simulink model "ASM_Traffic_A11"  (R2026a)
settings: Solver=ode1  StartTime=SIM.tstart.v  StopTime=SIM.tend.v  FixedStep=SIM.StepSize.v
PostLoadFcn:
  | if any(exist('dsrtsu_mdlpostloadfcn', 'file') ~= 0), dsrtsu_mdlpostloadfcn('Execute', bdroot); end
  | try, asm_mdl_postloadfcn(bdroot, 'UpdateModel', 3600); catch, disp(lasterr); end,
InitFcn:
  | , if any(exist('rtifpga_mdlclblib', 'file') ~= 0), rtifpga_mdlclblib('Init', bdroot); end,
  | , if any(exist('dsmpb_private', 'file') ~= 0), dsmpb_private('dsmpb_mdlclblib', 'Init', bdroot); end,
undefined symbols (not defined in the file): _to_, a0b2, ASM_BrakeHydraulics_DemoSystems, ASM_VehicleDynamics_DemoSystems, b98103fe8ad365046cd0, BrakeCircuit, controllerConfig, CPT, Crankshaft, DiscIntNeverNeededParam, dsmsi, FinalDriveAssembly, instance, MDL, ModeSignals, mu, Pos_BrakePedal_Maneuver, rad, RefSignals, s_to_rpm, SIM, SoftECU, Suspension, Tire, Transmission
libraries: ASM_Traffic_lib x135, simulink x98, ASM_Utils_lib x77, ASM_VehicleDynamics_lib x70, ASM_Environment_lib x22, dsmpblib x20, dsmsilib x15, MDLD_Utils_lib x10, ASM_BrakeHydraulics_lib x3, sl_discontinuities x2
(part 13 of 63)

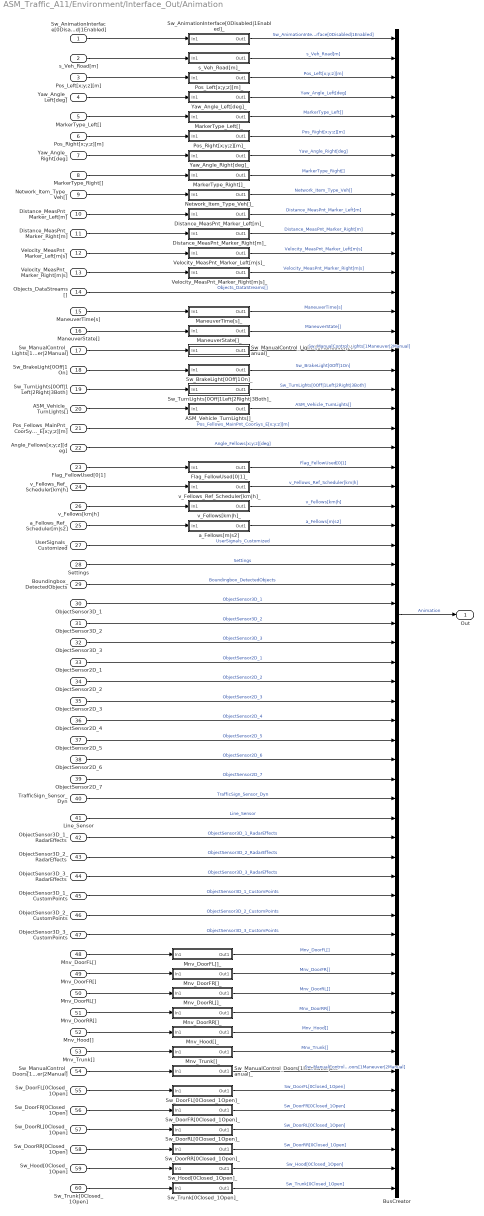
== system ASM_Traffic_A11/Environment/Interface_Out/Animation ==
  Sw_AnimationInterface[0Disabled|1Enabled] : Inport
  s_Veh_Road[m] : Inport  Port=2
  Pos_Left[x;y;z][m] : Inport  Port=3
  Yaw_Angle_Left[deg] : Inport  Port=4
  MarkerType_Left[] : Inport  Port=5
  Pos_Right[x;y;z][m] : Inport  Port=6
  Yaw_Angle_Right[deg] : Inport  Port=7
  MarkerType_Right[] : Inport  Port=8
  Network_Item_Type_Veh[] : Inport  Port=9
  Distance_MeasPnt_Marker_Left[m] : Inport  Port=10
  Distance_MeasPnt_Marker_Right[m] : Inport  Port=11
  Velocity_MeasPnt_Marker_Left[m|s] : Inport  Port=12
  Velocity_MeasPnt_Marker_Right[m|s] : Inport  Port=13
  Objects_DataStreams[] : Inport  Port=14
  ManeuverTime[s] : Inport  Port=15
  ManeuverState[] : Inport  Port=16
  Sw_ManualControl_Lights[1Maneuver|2Manual] : Inport  Port=17
  Sw_BrakeLight[0Off|1On] : Inport  Port=18
  Sw_TurnLights[0Off|1Left|2Right|3Both] : Inport  Port=19
  ASM_Vehicle_TurnLights[] : Inport  Port=20
  Pos_Fellows_MainPnt_CoorSys_E[x;y;z][m] : Inport  Port=21
  Angle_Fellows[x;y;z][deg] : Inport  Port=22
  Flag_FellowUsed[0|1] : Inport  Port=23
  v_Fellows_Ref_Scheduler[km|h] : Inport  Port=24
  a_Fellows_Ref_Scheduler[m|s2] : Inport  Port=25
  v_Fellows[km|h] : Inport  Port=26
  UserSignals_Customized : Inport  Port=27
  Settings : Inport  Port=28
  Boundingbox_DetectedObjects : Inport  Port=29
  ObjectSensor3D_1 : Inport  Port=30
  ObjectSensor3D_2 : Inport  Port=31
  ObjectSensor3D_3 : Inport  Port=32
  ObjectSensor2D_1 : Inport  Port=33
  ObjectSensor2D_2 : Inport  Port=34
  ObjectSensor2D_3 : Inport  Port=35
  ObjectSensor2D_4 : Inport  Port=36
  ObjectSensor2D_5 : Inport  Port=37
  ObjectSensor2D_6 : Inport  Port=38
  ObjectSensor2D_7 : Inport  Port=39
  TrafficSign_Sensor_Dyn : Inport  Port=40
  Line_Sensor : Inport  Port=41
  ObjectSensor3D_1_RadarEffects : Inport  Port=42
  ObjectSensor3D_2_RadarEffects : Inport  Port=43
  ObjectSensor3D_3_RadarEffects : Inport  Port=44
  ObjectSensor3D_1_CustomPoints : Inport  Port=45
  ObjectSensor3D_2_CustomPoints : Inport  Port=46
  ObjectSensor3D_3_CustomPoints : Inport  Port=47
  Mnv_DoorFL[] : Inport  Port=48
  Mnv_DoorFR[] : Inport  Port=49
  Mnv_DoorRL[] : Inport  Port=50
  Mnv_DoorRR[] : Inport  Port=51
  Mnv_Hood[] : Inport  Port=52
  Mnv_Trunk[] : Inport  Port=53
  Sw_ManualControl_Doors[1Maneuver|2Manual] : Inport  Port=54
  Sw_DoorFL[0Closed_1Open] : Inport  Port=55
  Sw_DoorFR[0Closed_1Open] : Inport  Port=56
  Sw_DoorRL[0Closed_1Open] : Inport  Port=57
  Sw_DoorRR[0Closed_1Open] : Inport  Port=58
  Sw_Hood[0Closed_1Open] : Inport  Port=59
  Sw_Trunk[0Closed_1Open] : Inport  Port=60
  ASM_Vehicle_TurnLights[]_ : Subsystem
      mask Display: disp('')
  BusCreator : BusCreator  Inputs=60
  Distance_MeasPnt_Marker_Left[m]_ : Subsystem
      mask Display: disp('')
  Distance_MeasPnt_Marker_Right[m]_ : Subsystem
      mask Display: disp('')
  Flag_FellowUsed[0|1]_ : Subsystem
      mask Display: disp('')
  ManeuverState[]_ : Subsystem
      mask Display: disp('')
  ManeuverTime[s]_ : Subsystem
      mask Display: disp('')
  MarkerType_Left[]_ : Subsystem
      mask Display: disp('')
  MarkerType_Right[]_ : Subsystem
      mask Display: disp('')
  Mnv_DoorFL[]_ : Subsystem
      mask Display: disp('')
  Mnv_DoorFR[]_ : Subsystem
      mask Display: disp('')
  Mnv_DoorRL[]_ : Subsystem
      mask Display: disp('')
  Mnv_DoorRR[]_ : Subsystem
      mask Display: disp('')
  Mnv_Hood[]_ : Subsystem
      mask Display: disp('')
  Mnv_Trunk[]_ : Subsystem
      mask Display: disp('')
  Network_Item_Type_Veh[]_ : Subsystem
      mask Display: disp('')
  Pos_Left[x;y;z][m]_ : Subsystem
      mask Display: disp('')
  Pos_Right[x;y;z][m]_ : Subsystem
      mask Display: disp('')
  Sw_AnimationInterface[0Disabled|1Enabled]_ : Subsystem
      mask Display: disp('')
  Sw_BrakeLight[0Off|1On]_ : Subsystem
      mask Display: disp('')
  Sw_DoorFL[0Closed_1Open]_ : Subsystem
      mask Display: disp('')
  Sw_DoorFR[0Closed_1Open]_ : Subsystem
      mask Display: disp('')
  Sw_DoorRL[0Closed_1Open]_ : Subsystem
      mask Display: disp('')
  Sw_DoorRR[0Closed_1Open]_ : Subsystem
      mask Display: disp('')
  Sw_Hood[0Closed_1Open]_ : Subsystem
      mask Display: disp('')
  Sw_ManualControl_Doors[1Maneuver|2Manual]_ : Subsystem
      mask Display: disp('')
  Sw_ManualControl_Lights[1Maneuver|2Manual]_ : Subsystem
      mask Display: disp('')
  Sw_Trunk[0Closed_1Open]_ : Subsystem
      mask Display: disp('')
  Sw_TurnLights[0Off|1Left|2Right|3Both]_ : Subsystem
      mask Display: disp('')
  Velocity_MeasPnt_Marker_Left[m|s]_ : Subsystem
      mask Display: disp('')
  Velocity_MeasPnt_Marker_Right[m|s]_ : Subsystem
      mask Display: disp('')
  Yaw_Angle_Left[deg]_ : Subsystem
      mask Display: disp('')
  Yaw_Angle_Right[deg]_ : Subsystem
      mask Display: disp('')
  a_Fellows[m|s2] : Subsystem
      mask Display: disp('')
  s_Veh_Road[m]_ : Subsystem
      mask Display: disp('')
  v_Fellows[km|h]_ : Subsystem
      mask Display: disp('')
  v_Fellows_Ref_Scheduler[km|h]_ : Subsystem
      mask Display: disp('')
  Out : Outport  VectorParamsAs1DForOutWhenUnconnected=off
  wires:
  Sw_AnimationInterface[0Disabled|1Enabled]_/1(Out1) -> BusCreator/1  "Sw_AnimationInterface[0Disabled|1Enabled]"
  Sw_AnimationInterface[0Disabled|1Enabled]/1 -> Sw_AnimationInterface[0Disabled|1Enabled]_/1(In1)
  a_Fellows[m|s2]/1(Out1) -> BusCreator/26  "a_Fellows[m|s2]"
  a_Fellows_Ref_Scheduler[m|s2]/1 -> a_Fellows[m|s2]/1(In1)
  ObjectSensor2D_1/1 -> BusCreator/33  "ObjectSensor2D_1"
  ObjectSensor2D_2/1 -> BusCreator/34  "ObjectSensor2D_2"
  ObjectSensor3D_1/1 -> BusCreator/30  "ObjectSensor3D_1"
  ObjectSensor2D_3/1 -> BusCreator/35  "ObjectSensor2D_3"
  ObjectSensor3D_2/1 -> BusCreator/31  "ObjectSensor3D_2"
  ObjectSensor2D_6/1 -> BusCreator/38  "ObjectSensor2D_6"
  ObjectSensor2D_4/1 -> BusCreator/36  "ObjectSensor2D_4"
  ObjectSensor2D_7/1 -> BusCreator/39  "ObjectSensor2D_7"
  TrafficSign_Sensor_Dyn/1 -> BusCreator/40  "TrafficSign_Sensor_Dyn"
  ObjectSensor3D_3_CustomPoints/1 -> BusCreator/47  "ObjectSensor3D_3_CustomPoints"
  ObjectSensor3D_3/1 -> BusCreator/32  "ObjectSensor3D_3"
  ObjectSensor3D_1_RadarEffects/1 -> BusCreator/42  "ObjectSensor3D_1_RadarEffects"
  ObjectSensor3D_3_RadarEffects/1 -> BusCreator/44  "ObjectSensor3D_3_RadarEffects"
  ObjectSensor3D_2_CustomPoints/1 -> BusCreator/46  "ObjectSensor3D_2_CustomPoints"
  ObjectSensor2D_5/1 -> BusCreator/37  "ObjectSensor2D_5"
  Line_Sensor/1 -> BusCreator/41  "Line_Sensor"
  ObjectSensor3D_1_CustomPoints/1 -> BusCreator/45  "ObjectSensor3D_1_CustomPoints"
  ObjectSensor3D_2_RadarEffects/1 -> BusCreator/43  "ObjectSensor3D_2_RadarEffects"
  Boundingbox_DetectedObjects/1 -> BusCreator/29  "Boundingbox_DetectedObjects"
  v_Fellows[km|h]_/1(Out1) -> BusCreator/25  "v_Fellows[km|h]"
  v_Fellows_Ref_Scheduler[km|h]_/1(Out1) -> BusCreator/24  "v_Fellows_Ref_Scheduler[km|h]"
  Flag_FellowUsed[0|1]_/1(Out1) -> BusCreator/23  "Flag_FellowUsed[0|1]"
  Pos_Fellows_MainPnt_CoorSys_E[x;y;z][m]/1 -> BusCreator/21  "Pos_Fellows_MainPnt_CoorSys_E[x;y;z][m]"
  Settings/1 -> BusCreator/28  "Settings"
  v_Fellows_Ref_Scheduler[km|h]/1 -> v_Fellows_Ref_Scheduler[km|h]_/1(In1)
  UserSignals_Customized/1 -> BusCreator/27  "UserSignals_Customized"
  Angle_Fellows[x;y;z][deg]/1 -> BusCreator/22  "Angle_Fellows[x;y;z][deg]"
  v_Fellows[km|h]/1 -> v_Fellows[km|h]_/1(In1)
  Flag_FellowUsed[0|1]/1 -> Flag_FellowUsed[0|1]_/1(In1)
  ASM_Vehicle_TurnLights[]_/1(Out1) -> BusCreator/20  "ASM_Vehicle_TurnLights[]"
  Sw_TurnLights[0Off|1Left|2Right|3Both]_/1(Out1) -> BusCreator/19  "Sw_TurnLights[0Off|1Left|2Right|3Both]"
  Sw_BrakeLight[0Off|1On]_/1(Out1) -> BusCreator/18  "Sw_BrakeLight[0Off|1On]"
  Sw_ManualControl_Lights[1Maneuver|2Manual]_/1(Out1) -> BusCreator/17  "Sw_ManualControl_Lights[1Maneuver|2Manual]"
  ManeuverState[]_/1(Out1) -> BusCreator/16  "ManeuverState[]"
  ManeuverTime[s]_/1(Out1) -> BusCreator/15  "ManeuverTime[s]"
  ManeuverState[]/1 -> ManeuverState[]_/1(In1)
  Sw_BrakeLight[0Off|1On]/1 -> Sw_BrakeLight[0Off|1On]_/1(In1)
  ManeuverTime[s]/1 -> ManeuverTime[s]_/1(In1)
  Sw_TurnLights[0Off|1Left|2Right|3Both]/1 -> Sw_TurnLights[0Off|1Left|2Right|3Both]_/1(In1)
  Sw_ManualControl_Lights[1Maneuver|2Manual]/1 -> Sw_ManualControl_Lights[1Maneuver|2Manual]_/1(In1)
  ASM_Vehicle_TurnLights[]/1 -> ASM_Vehicle_TurnLights[]_/1(In1)
  Objects_DataStreams[]/1 -> BusCreator/14  "Objects_DataStreams[]"
  Velocity_MeasPnt_Marker_Right[m|s]_/1(Out1) -> BusCreator/13  "Velocity_MeasPnt_Marker_Right[m|s]"
  Velocity_MeasPnt_Marker_Left[m|s]_/1(Out1) -> BusCreator/12  "Velocity_MeasPnt_Marker_Left[m|s]"
  Distance_MeasPnt_Marker_Right[m]_/1(Out1) -> BusCreator/11  "Distance_MeasPnt_Marker_Right[m]"
  Distance_MeasPnt_Marker_Left[m]_/1(Out1) -> BusCreator/10  "Distance_MeasPnt_Marker_Left[m]"
  Network_Item_Type_Veh[]_/1(Out1) -> BusCreator/9  "Network_Item_Type_Veh[]"
  MarkerType_Right[]_/1(Out1) -> BusCreator/8  "MarkerType_Right[]"
  Yaw_Angle_Right[deg]_/1(Out1) -> BusCreator/7  "Yaw_Angle_Right[deg]"
  Pos_Right[x;y;z][m]_/1(Out1) -> BusCreator/6  "Pos_Right[x;y;z][m]"
  MarkerType_Left[]_/1(Out1) -> BusCreator/5  "MarkerType_Left[]"
  Yaw_Angle_Left[deg]_/1(Out1) -> BusCreator/4  "Yaw_Angle_Left[deg]"
  Pos_Left[x;y;z][m]_/1(Out1) -> BusCreator/3  "Pos_Left[x;y;z][m]"
  s_Veh_Road[m]_/1(Out1) -> BusCreator/2  "s_Veh_Road[m]"
  s_Veh_Road[m]/1 -> s_Veh_Road[m]_/1(In1)
  Pos_Left[x;y;z][m]/1 -> Pos_Left[x;y;z][m]_/1(In1)
  Pos_Right[x;y;z][m]/1 -> Pos_Right[x;y;z][m]_/1(In1)
  Yaw_Angle_Left[deg]/1 -> Yaw_Angle_Left[deg]_/1(In1)
  Distance_MeasPnt_Marker_Right[m]/1 -> Distance_MeasPnt_Marker_Right[m]_/1(In1)
  MarkerType_Left[]/1 -> MarkerType_Left[]_/1(In1)
  MarkerType_Right[]/1 -> MarkerType_Right[]_/1(In1)
  Yaw_Angle_Right[deg]/1 -> Yaw_Angle_Right[deg]_/1(In1)
  Velocity_MeasPnt_Marker_Right[m|s]/1 -> Velocity_MeasPnt_Marker_Right[m|s]_/1(In1)
  Network_Item_Type_Veh[]/1 -> Network_Item_Type_Veh[]_/1(In1)
  Velocity_MeasPnt_Marker_Left[m|s]/1 -> Velocity_MeasPnt_Marker_Left[m|s]_/1(In1)
  Distance_MeasPnt_Marker_Left[m]/1 -> Distance_MeasPnt_Marker_Left[m]_/1(In1)
  BusCreator/1 -> Out/1  "Animation"
  Mnv_Trunk[]/1 -> Mnv_Trunk[]_/1(In1)
  Mnv_DoorFR[]/1 -> Mnv_DoorFR[]_/1(In1)
  Mnv_Hood[]/1 -> Mnv_Hood[]_/1(In1)
  Mnv_DoorRL[]/1 -> Mnv_DoorRL[]_/1(In1)
  Mnv_DoorRR[]/1 -> Mnv_DoorRR[]_/1(In1)
  Mnv_DoorFL[]_/1(Out1) -> BusCreator/48  "Mnv_DoorFL[]"
  Mnv_DoorFL[]/1 -> Mnv_DoorFL[]_/1(In1)
  Mnv_DoorFR[]_/1(Out1) -> BusCreator/49  "Mnv_DoorFR[]"
  Mnv_DoorRL[]_/1(Out1) -> BusCreator/50  "Mnv_DoorRL[]"
  Mnv_DoorRR[]_/1(Out1) -> BusCreator/51  "Mnv_DoorRR[]"
  Mnv_Hood[]_/1(Out1) -> BusCreator/52  "Mnv_Hood[]"
  Mnv_Trunk[]_/1(Out1) -> BusCreator/53  "Mnv_Trunk[]"
  Sw_DoorFL[0Closed_1Open]_/1(Out1) -> BusCreator/55  "Sw_DoorFL[0Closed_1Open]"
  Sw_DoorFR[0Closed_1Open]_/1(Out1) -> BusCreator/56  "Sw_DoorFR[0Closed_1Open]"
  Sw_ManualControl_Doors[1Maneuver|2Manual]_/1(Out1) -> BusCreator/54  "Sw_ManualControl_Doors[1Maneuver|2Manual]"
  Sw_Hood[0Closed_1Open]_/1(Out1) -> BusCreator/59  "Sw_Hood[0Closed_1Open]"
  Sw_DoorRR[0Closed_1Open]_/1(Out1) -> BusCreator/58  "Sw_DoorRR[0Closed_1Open]"
  Sw_DoorRL[0Closed_1Open]_/1(Out1) -> BusCreator/57  "Sw_DoorRL[0Closed_1Open]"
  Sw_Trunk[0Closed_1Open]_/1(Out1) -> BusCreator/60  "Sw_Trunk[0Closed_1Open]"
  Sw_ManualControl_Doors[1Maneuver|2Manual]/1 -> Sw_ManualControl_Doors[1Maneuver|2Manual]_/1(In1)
  Sw_DoorFL[0Closed_1Open]/1 -> Sw_DoorFL[0Closed_1Open]_/1(In1)
  Sw_DoorFR[0Closed_1Open]/1 -> Sw_DoorFR[0Closed_1Open]_/1(In1)
  Sw_DoorRL[0Closed_1Open]/1 -> Sw_DoorRL[0Closed_1Open]_/1(In1)
  Sw_DoorRR[0Closed_1Open]/1 -> Sw_DoorRR[0Closed_1Open]_/1(In1)
  Sw_Hood[0Closed_1Open]/1 -> Sw_Hood[0Closed_1Open]_/1(In1)
  Sw_Trunk[0Closed_1Open]/1 -> Sw_Trunk[0Closed_1Open]_/1(In1)

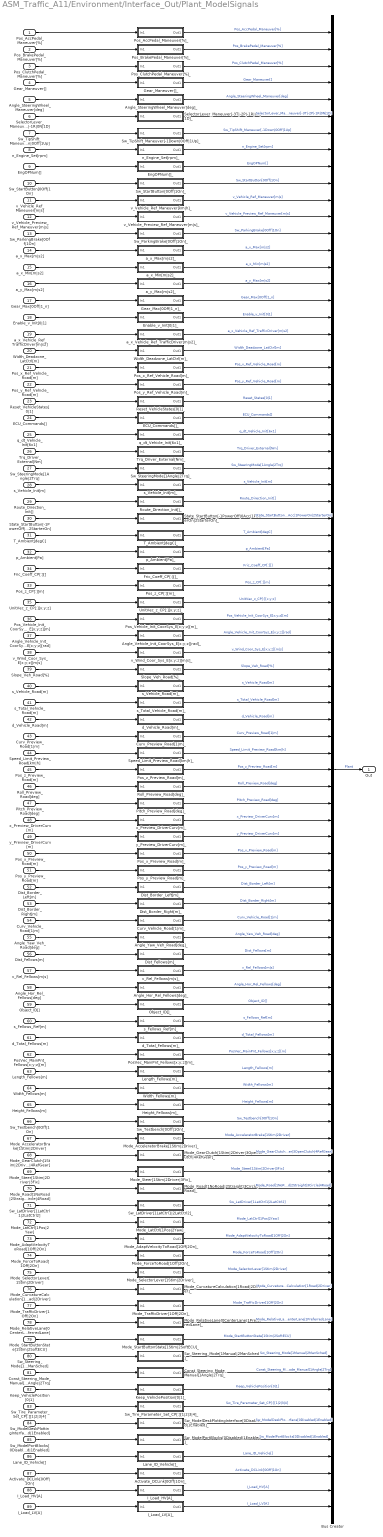
== system ASM_Traffic_A11/Environment/Interface_Out/Plant_ModelSignals ==
  Pos_AccPedal_Maneuver[%] : Inport
  Pos_BrakePedal_Maneuver[%] : Inport  Port=2
  Pos_ClutchPedal_Maneuver[%] : Inport  Port=3
  Gear_Maneuver[] : Inport  Port=4
  Angle_SteeringWheel_Maneuver[deg] : Inport  Port=5
  SelectorLever_Maneuver[-3T|-2P|-1R|0N|1D] : Inport  Port=6
  Sw_TipShift_Maneuver[-1Down|0Off|1Up] : Inport  Port=7
  n_Engine_Set[rpm] : Inport  Port=8
  EngOPNum[] : Inport  Port=9
  Sw_StartButton[0Off|1On] : Inport  Port=10
  v_Vehicle_Ref_Maneuver[m|s] : Inport  Port=11
  v_Vehicle_Preview_Ref_Maneuver[m|s] : Inport  Port=12
  Sw_ParkingBrake[0Off|1On] : Inport  Port=13
  a_x_Max[m|s2] : Inport  Port=14
  a_x_Min[m|s2] : Inport  Port=15
  a_y_Max[m|s2] : Inport  Port=16
  Gear_Max[0Off|1_n] : Inport  Port=17
  Enable_v_Init[0|1] : Inport  Port=18
  a_x_Vehicle_Ref_TrafficDriver[m|s2] : Inport  Port=19
  Width_Deadzone_LatCtrl[m] : Inport  Port=20
  Pos_x_Ref_Vehicle_Road[m] : Inport  Port=21
  Pos_y_Ref_Vehicle_Road[m] : Inport  Port=22
  Reset_VehicleStates[0|1] : Inport  Port=23
  ECU_Commands[] : Inport  Port=24
  q_dt_Vehicle_Init[6x1] : Inport  Port=25
  Trq_Driver_External[Nm] : Inport  Port=26
  Sw_SteeringMode[1Angle|2Trq] : Inport  Port=27
  s_Vehicle_Init[m] : Inport  Port=28
  Route_Direction_Init[] : Inport  Port=29
  State_StartButton[-1PowerOff|0Acc|1PowerOn|2StarterOn] : Inport  Port=30
  T_Ambient[degC] : Inport  Port=31
  p_Ambient[Pa] : Inport  Port=32
  Pos_z_CP[:][m] : Inport  Port=33
  Fric_Coeff_CP[:][] : Inport  Port=34
  UnitVec_z_CP[:][x;y;z] : Inport  Port=35
  Pos_Vehicle_Init_CoorSys_E[x;y;z][m] : Inport  Port=36
  Angle_Vehicle_Init_CoorSys_E[x;y;z][rad] : Inport  Port=37
  v_Wind_Coor_Sys_E[x;y;z][m|s] : Inport  Port=38
  Slope_Veh_Road[%] : Inport  Port=39
  s_Vehicle_Road[m] : Inport  Port=40
  s_Total_Vehicle_Road[m] : Inport  Port=41
  d_Vehicle_Road[m] : Inport  Port=42
  Curv_Preview_Road[1|m] : Inport  Port=43
  Speed_Limit_Preview_Road[km|h] : Inport  Port=44
  Pos_z_Preview_Road[m] : Inport  Port=45
  Roll_Preview_Road[deg] : Inport  Port=46
  Pitch_Preview_Road[deg] : Inport  Port=47
  x_Preview_DriverCurv[m] : Inport  Port=48
  y_Preview_DriverCurv[m] : Inport  Port=49
  Pos_x_Preview_Road[m] : Inport  Port=50
  Pos_y_Preview_Road[m] : Inport  Port=51
  Dist_Border_Left[m] : Inport  Port=52
  Dist_Border_Right[m] : Inport  Port=53
  Curv_Vehicle_Road[1|m] : Inport  Port=54
  Angle_Yaw_Veh_Road[deg] : Inport  Port=55
  Dist_Fellows[m] : Inport  Port=56
  v_Rel_Fellows[m|s] : Inport  Port=57
  Angle_Hor_Rel_Fellows[deg] : Inport  Port=58
  Object_ID[] : Inport  Port=59
  s_Fellows_Ref[m] : Inport  Port=60
  d_Total_Fellows[m] : Inport  Port=61
  PosVec_MainPnt_Fellows[x;y;z][m] : Inport  Port=62
  Length_Fellows[m] : Inport  Port=63
  Width_Fellows[m] : Inport  Port=64
  Height_Fellows[m] : Inport  Port=65
  Sw_Testbench[0Off|1On] : Inport  Port=66
  Mode_AcceleratorBrake[1Stim|2Driver] : Inport  Port=67
  Mode_GearClutch[1Stim|2Driver|3OpenClutch|4RefGear] : Inport  Port=68
  Mode_Steer[1Stim|2Driver|3Fix] : Inport  Port=69
  Mode_Road[1NoRoad|2Straight|3Circle|4Road] : Inport  Port=70
  Sw_LatDriver[1LatCtrl1|2LatCtrl2] : Inport  Port=71
  Mode_LatCtrl[1Pos|2Yaw] : Inport  Port=72
  Mode_AdaptVelocityToRoad[1Off|2On] : Inport  Port=73
  Mode_ForceToRoad[1Off|2On] : Inport  Port=74
  Mode_SelectorLever[1Stim|2Driver] : Inport  Port=75
  Mode_CurvatureCalculation[1Road|2Driver] : Inport  Port=76
  Mode_TrafficDriver[1Off|2On] : Inport  Port=77
  Mode_RelativeLane[0CenterLane|1PreferredLane] : Inport  Port=78
  Mode_StartButtonState[1Stim|2SoftECU] : Inport  Port=79
  Sw_Steering_Mode[1Manual|2ManSched] : Inport  Port=80
  Const_Steering_Mode_Manual[1Angle|2Trq] : Inport  Port=81
  Keep_VehiclePosition[0|1] : Inport  Port=82
  Sw_Tire_Parameter_Set_CP[:][1|2|3|4] : Inport  Port=83
  Sw_ModelDeskPlottingInterface[0Disabled|1Enabled] : Inport  Port=84
  Sw_ModelPortBlocks[0Disabled|1Enabled] : Inport  Port=85
  Lane_ID_Vehicle[] : Inport  Port=86
  Activate_DCLink[0Off|1On] : Inport  Port=87
  I_Load_HV[A] : Inport  Port=88
  I_Load_LV[A] : Inport  Port=89
  Activate_DCLink[0Off|1On]_ : Subsystem
      mask Display: disp('')
  Angle_Hor_Rel_Fellows[deg]_ : Subsystem
      mask Display: disp('')
  Angle_SteeringWheel_Maneuver[deg]_ : Subsystem
      mask Display: disp('')
  Angle_Vehicle_Init_CoorSys_E[x;y;z][rad]_ : Subsystem
      mask Display: disp('')
  Angle_Yaw_Veh_Road[deg]_ : Subsystem
      mask Display: disp('')
  Bus Creator : BusCreator  Inputs=89
  Const_Steering_Mode_Manual[1Angle|2Trq]_ : Subsystem
      mask Display: disp('')
  Curv_Preview_Road[1|m]_ : Subsystem
      mask Display: disp('')
  Curv_Vehicle_Road[1|m]_ : Subsystem
      mask Display: disp('')
  Dist_Border_Left[m]_ : Subsystem
      mask Display: disp('')
  Dist_Border_Right[m]_ : Subsystem
      mask Display: disp('')
  Dist_Fellows[m]_ : Subsystem
      mask Display: disp('')
  ECU_Commands[]_ : Subsystem
      mask Display: disp('')
  Enable_v_Init[0|1]_ : Subsystem
      mask Display: disp('')
  EngOPNum[]_ : Subsystem
      mask Display: disp('')
  Fric_Coeff_CP[:][]_ : Subsystem
      mask Display: disp('')
  Gear_Maneuver[]_ : Subsystem
      mask Display: disp('')
  Gear_Max[0Off|1_n]_ : Subsystem
      mask Display: disp('')
  Height_Fellows[m]_ : Subsystem
      mask Display: disp('')
  I_Load_HV[A]_ : Subsystem
      mask Display: disp('')
  I_Load_LV[A]_ : Subsystem
      mask Display: disp('')
  Keep_VehiclePosition[0|1]_ : Subsystem
      mask Display: disp('')
  Lane_ID_Vehicle[]_ : Subsystem
      mask Display: disp('')
  Length_Fellows[m]_ : Subsystem
      mask Display: disp('')
  Mode_AcceleratorBrake[1Stim|2Driver]_ : Subsystem
      mask Display: disp('')
  Mode_AdaptVelocityToRoad[1Off|2On]_ : Subsystem
      mask Display: disp('')
  Mode_CurvatureCalculation[1Road|2Driver]_ : Subsystem
      mask Display: disp('')
  Mode_ForceToRoad[1Off|2On]_ : Subsystem
      mask Display: disp('')
  Mode_GearClutch[1Stim|2Driver|3OpenClutch|4RefGear]_ : Subsystem
      mask Display: disp('')
  Mode_LatCtrl[1Pos|2Yaw]_ : Subsystem
      mask Display: disp('')
  Mode_RelativeLane[0CenterLane|1PreferredLane]_ : Subsystem
      mask Display: disp('')
  Mode_Road[1NoRoad|2Straight|3Circle|4Road]_ : Subsystem
      mask Display: disp('')
  Mode_SelectorLever[1Stim|2Driver]_ : Subsystem
      mask Display: disp('')
  Mode_StartButtonState[1Stim|2SoftECU]_ : Subsystem
      mask Display: disp('')
  Mode_Steer[1Stim|2Driver|3Fix]_ : Subsystem
      mask Display: disp('')
  Mode_TrafficDriver[1Off|2On]_ : Subsystem
      mask Display: disp('')
  Object_ID[]_ : Subsystem
      mask Display: disp('')
  Pitch_Preview_Road[deg]_ : Subsystem
      mask Display: disp('')
  PosVec_MainPnt_Fellows[x;y;z][m]_ : Subsystem
      mask Display: disp('')
  Pos_AccPedal_Maneuver[%]_ : Subsystem
      mask Display: disp('')
  Pos_BrakePedal_Maneuver[%]_ : Subsystem
      mask Display: disp('')
  Pos_ClutchPedal_Maneuver[%]_ : Subsystem
      mask Display: disp('')
  Pos_Vehicle_Init_CoorSys_E[x;y;z][m]_ : Subsystem
      mask Display: disp('')
  Pos_x_Preview_Road[m]_ : Subsystem
      mask Display: disp('')
  Pos_x_Ref_Vehicle_Road[m]_ : Subsystem
      mask Display: disp('')
  Pos_y_Preview_Road[m]_ : Subsystem
      mask Display: disp('')
  Pos_y_Ref_Vehicle_Road[m]_ : Subsystem
      mask Display: disp('')
  Pos_z_CP[:][m]_ : Subsystem
      mask Display: disp('')
  Pos_z_Preview_Road[m]_ : Subsystem
      mask Display: disp('')
  Reset_VehicleStates[0|1]_ : Subsystem
      mask Display: disp('')
  Roll_Preview_Road[deg]_ : Subsystem
      mask Display: disp('')
  Route_Direction_Init[]_ : Subsystem
      mask Display: disp('')
  SelectorLever_Maneuver[-3T|-2P|-1R|0N|1D]_ : Subsystem
      mask Display: disp('')
  Slope_Veh_Road[%]_ : Subsystem
      mask Display: disp('')
  Speed_Limit_Preview_Road[km|h]_ : Subsystem
      mask Display: disp('')
  State_StartButton[-1PowerOff|0Acc|1PowerOn|2StarterOn]_ : Subsystem
      mask Display: disp('')
  Sw_LatDriver[1LatCtrl1|2LatCtrl2]_ : Subsystem
      mask Display: disp('')
  Sw_ModelDeskPlottingInterface[0Disabled|1Enabled]_ : Subsystem
      mask Display: disp('')
  Sw_ModelPortBlocks[0Disabled|1Enabled]_ : Subsystem
      mask Display: disp('')
  Sw_ParkingBrake[0Off|1On]_ : Subsystem
      mask Display: disp('')
  Sw_StartButton[0Off|1On]_ : Subsystem
      mask Display: disp('')
  Sw_SteeringMode[1Angle|2Trq]_ : Subsystem
      mask Display: disp('')
  Sw_Steering_Mode[1Manual|2ManSched]_ : Subsystem
      mask Display: disp('')
  Sw_Testbench[0Off|1On]_ : Subsystem
      mask Display: disp('')
  Sw_TipShift_Maneuver[-1Down|0Off|1Up]_ : Subsystem
      mask Display: disp('')
  Sw_Tire_Parameter_Set_CP[:][1|2|3|4]_ : Subsystem
      mask Display: disp('')
  T_Ambient[degC]_ : Subsystem
      mask Display: disp('')
  Trq_Driver_External[Nm]_ : Subsystem
      mask Display: disp('')
  UnitVec_z_CP[:][x;y;z]_ : Subsystem
      mask Display: disp('')
  Width_Deadzone_LatCtrl[m]_ : Subsystem
      mask Display: disp('')
  Width_Fellows[m]_ : Subsystem
      mask Display: disp('')
  a_x_Max[m|s2]_ : Subsystem
      mask Display: disp('')
  a_x_Min[m|s2]_ : Subsystem
      mask Display: disp('')
  a_x_Vehicle_Ref_TrafficDriver[m|s2]_ : Subsystem
      mask Display: disp('')
  a_y_Max[m|s2]_ : Subsystem
      mask Display: disp('')
  d_Total_Fellows[m]_ : Subsystem
      mask Display: disp('')
  d_Vehicle_Road[m]_ : Subsystem
      mask Display: disp('')
  n_Engine_Set[rpm]_ : Subsystem
      mask Display: disp('')
  p_Ambient[Pa]_ : Subsystem
      mask Display: disp('')
  q_dt_Vehicle_Init[6x1]_ : Subsystem
      mask Display: disp('')
  s_Fellows_Ref[m]_ : Subsystem
      mask Display: disp('')
  s_Total_Vehicle_Road[m]_ : Subsystem
      mask Display: disp('')
  s_Vehicle_Init[m]_ : Subsystem
      mask Display: disp('')
  s_Vehicle_Road[m]_ : Subsystem
      mask Display: disp('')
  v_Rel_Fellows[m|s]_ : Subsystem
      mask Display: disp('')
  v_Vehicle_Preview_Ref_Maneuver[m|s]_ : Subsystem
      mask Display: disp('')
  v_Vehicle_Ref_Maneuver[km|h]_ : Subsystem
      mask Display: disp('')
  v_Wind_Coor_Sys_E[x;y;z][m|s]_ : Subsystem
      mask Display: disp('')
  x_Preview_DriverCurv[m]_ : Subsystem
      mask Display: disp('')
  y_Preview_DriverCurv[m]_ : Subsystem
      mask Display: disp('')
  Out : Outport  VectorParamsAs1DForOutWhenUnconnected=off
  wires:
  Lane_ID_Vehicle[]_/1(Out1) -> Bus Creator/86  "Lane_ID_Vehicle[]"
  Lane_ID_Vehicle[]/1 -> Lane_ID_Vehicle[]_/1(In1)
  Sw_ModelDeskPlottingInterface[0Disabled|1Enabled]/1 -> Sw_ModelDeskPlottingInterface[0Disabled|1Enabled]_/1(In1)
  Sw_ModelDeskPlottingInterface[0Disabled|1Enabled]_/1(Out1) -> Bus Creator/84  "Sw_ModelDeskPlottingInterface[0Disabled|1Enabled]"
  Sw_ModelPortBlocks[0Disabled|1Enabled]/1 -> Sw_ModelPortBlocks[0Disabled|1Enabled]_/1(In1)
  Sw_ModelPortBlocks[0Disabled|1Enabled]_/1(Out1) -> Bus Creator/85  "Sw_ModelPortBlocks[0Disabled|1Enabled]"
  Bus Creator/1 -> Out/1  "Plant"
  Enable_v_Init[0|1]_/1(Out1) -> Bus Creator/18  "Enable_v_Init[0|1]"
  Enable_v_Init[0|1]/1 -> Enable_v_Init[0|1]_/1(In1)
  SelectorLever_Maneuver[-3T|-2P|-1R|0N|1D]/1 -> SelectorLever_Maneuver[-3T|-2P|-1R|0N|1D]_/1(In1)
  Sw_StartButton[0Off|1On]/1 -> Sw_StartButton[0Off|1On]_/1(In1)
  Gear_Max[0Off|1_n]/1 -> Gear_Max[0Off|1_n]_/1(In1)
  v_Vehicle_Preview_Ref_Maneuver[m|s]_/1(Out1) -> Bus Creator/12  "v_Vehicle_Preview_Ref_Maneuver[m|s]"
  v_Vehicle_Ref_Maneuver[km|h]_/1(Out1) -> Bus Creator/11  "v_Vehicle_Ref_Maneuver[m|s]"
  Pos_x_Ref_Vehicle_Road[m]/1 -> Pos_x_Ref_Vehicle_Road[m]_/1(In1)
  Gear_Max[0Off|1_n]_/1(Out1) -> Bus Creator/17  "Gear_Max[0Off|1_n]"
  Sw_StartButton[0Off|1On]_/1(Out1) -> Bus Creator/10  "Sw_StartButton[0Off|1On]"
  EngOPNum[]/1 -> EngOPNum[]_/1(In1)
  Sw_TipShift_Maneuver[-1Down|0Off|1Up]_/1(Out1) -> Bus Creator/7  "Sw_TipShift_Maneuver[-1Down|0Off|1Up]"
  n_Engine_Set[rpm]/1 -> n_Engine_Set[rpm]_/1(In1)
  Pos_BrakePedal_Maneuver[%]_/1(Out1) -> Bus Creator/2  "Pos_BrakePedal_Maneuver[%]"
  Pos_x_Ref_Vehicle_Road[m]_/1(Out1) -> Bus Creator/21  "Pos_x_Ref_Vehicle_Road[m]"
  Pos_ClutchPedal_Maneuver[%]_/1(Out1) -> Bus Creator/3  "Pos_ClutchPedal_Maneuver[%]"
  a_y_Max[m|s2]_/1(Out1) -> Bus Creator/16  "a_y_Max[m|s2]"
  a_x_Max[m|s2]/1 -> a_x_Max[m|s2]_/1(In1)
  Angle_SteeringWheel_Maneuver[deg]_/1(Out1) -> Bus Creator/5  "Angle_SteeringWheel_Maneuver[deg]"
  Sw_ParkingBrake[0Off|1On]/1 -> Sw_ParkingBrake[0Off|1On]_/1(In1)
  Pos_ClutchPedal_Maneuver[%]/1 -> Pos_ClutchPedal_Maneuver[%]_/1(In1)
  Gear_Maneuver[]/1 -> Gear_Maneuver[]_/1(In1)
  Angle_SteeringWheel_Maneuver[deg]/1 -> Angle_SteeringWheel_Maneuver[deg]_/1(In1)
  Pos_AccPedal_Maneuver[%]_/1(Out1) -> Bus Creator/1  "Pos_AccPedal_Maneuver[%]"
  a_x_Min[m|s2]/1 -> a_x_Min[m|s2]_/1(In1)
  v_Vehicle_Ref_Maneuver[m|s]/1 -> v_Vehicle_Ref_Maneuver[km|h]_/1(In1)
  Pos_AccPedal_Maneuver[%]/1 -> Pos_AccPedal_Maneuver[%]_/1(In1)
  a_y_Max[m|s2]/1 -> a_y_Max[m|s2]_/1(In1)
  v_Vehicle_Preview_Ref_Maneuver[m|s]/1 -> v_Vehicle_Preview_Ref_Maneuver[m|s]_/1(In1)
  SelectorLever_Maneuver[-3T|-2P|-1R|0N|1D]_/1(Out1) -> Bus Creator/6  "SelectorLever_Maneuver[-3T|-2P|-1R|0N|1D]"
  a_x_Max[m|s2]_/1(Out1) -> Bus Creator/14  "a_x_Max[m|s2]"
  Width_Deadzone_LatCtrl[m]/1 -> Width_Deadzone_LatCtrl[m]_/1(In1)
  Pos_BrakePedal_Maneuver[%]/1 -> Pos_BrakePedal_Maneuver[%]_/1(In1)
  a_x_Min[m|s2]_/1(Out1) -> Bus Creator/15  "a_x_Min[m|s2]"
  Gear_Maneuver[]_/1(Out1) -> Bus Creator/4  "Gear_Maneuver[]"
  a_x_Vehicle_Ref_TrafficDriver[m|s2]_/1(Out1) -> Bus Creator/19  "a_x_Vehicle_Ref_TrafficDriver[m|s2]"
  a_x_Vehicle_Ref_TrafficDriver[m|s2]/1 -> a_x_Vehicle_Ref_TrafficDriver[m|s2]_/1(In1)
  EngOPNum[]_/1(Out1) -> Bus Creator/9  "EngOPNum[]"
  Pos_y_Ref_Vehicle_Road[m]/1 -> Pos_y_Ref_Vehicle_Road[m]_/1(In1)
  Pos_y_Ref_Vehicle_Road[m]_/1(Out1) -> Bus Creator/22  "Pos_y_Ref_Vehicle_Road[m]"
  Sw_ParkingBrake[0Off|1On]_/1(Out1) -> Bus Creator/13  "Sw_ParkingBrake[0Off|1On]"
  Width_Deadzone_LatCtrl[m]_/1(Out1) -> Bus Creator/20  "Width_Deadzone_LatCtrl[m]"
  Sw_TipShift_Maneuver[-1Down|0Off|1Up]/1 -> Sw_TipShift_Maneuver[-1Down|0Off|1Up]_/1(In1)
  n_Engine_Set[rpm]_/1(Out1) -> Bus Creator/8  "n_Engine_Set[rpm]"
  State_StartButton[-1PowerOff|0Acc|1PowerOn|2StarterOn]_/1(Out1) -> Bus Creator/30  "State_StartButton[-1PowerOff|0Acc|1PowerOn|2StarterOn]"
  State_StartButton[-1PowerOff|0Acc|1PowerOn|2StarterOn]/1 -> State_StartButton[-1PowerOff|0Acc|1PowerOn|2StarterOn]_/1(In1)
  Angle_Yaw_Veh_Road[deg]/1 -> Angle_Yaw_Veh_Road[deg]_/1(In1)
  Angle_Yaw_Veh_Road[deg]_/1(Out1) -> Bus Creator/55  "Angle_Yaw_Veh_Road[deg]"
  Pos_y_Preview_Road[m]_/1(Out1) -> Bus Creator/51  "Pos_y_Preview_Road[m]"
  Pos_x_Preview_Road[m]_/1(Out1) -> Bus Creator/50  "Pos_x_Preview_Road[m]"
  Pos_x_Preview_Road[m]/1 -> Pos_x_Preview_Road[m]_/1(In1)
  Pos_y_Preview_Road[m]/1 -> Pos_y_Preview_Road[m]_/1(In1)
  Route_Direction_Init[]_/1(Out1) -> Bus Creator/29  "Route_Direction_Init[]"
  s_Vehicle_Init[m]_/1(Out1) -> Bus Creator/28  "s_Vehicle_Init[m]"
  Route_Direction_Init[]/1 -> Route_Direction_Init[]_/1(In1)
  s_Vehicle_Init[m]/1 -> s_Vehicle_Init[m]_/1(In1)
  Curv_Vehicle_Road[1|m]_/1(Out1) -> Bus Creator/54  "Curv_Vehicle_Road[1|m]"
  Curv_Vehicle_Road[1|m]/1 -> Curv_Vehicle_Road[1|m]_/1(In1)
  Dist_Border_Right[m]_/1(Out1) -> Bus Creator/53  "Dist_Border_Right[m]"
  Dist_Border_Left[m]_/1(Out1) -> Bus Creator/52  "Dist_Border_Left[m]"
  Dist_Border_Left[m]/1 -> Dist_Border_Left[m]_/1(In1)
  Dist_Border_Right[m]/1 -> Dist_Border_Right[m]_/1(In1)
  y_Preview_DriverCurv[m]_/1(Out1) -> Bus Creator/49  "y_Preview_DriverCurv[m]"
  x_Preview_DriverCurv[m]_/1(Out1) -> Bus Creator/48  "x_Preview_DriverCurv[m]"
  Pitch_Preview_Road[deg]_/1(Out1) -> Bus Creator/47  "Pitch_Preview_Road[deg]"
  Roll_Preview_Road[deg]_/1(Out1) -> Bus Creator/46  "Roll_Preview_Road[deg]"
  Pos_z_Preview_Road[m]_/1(Out1) -> Bus Creator/45  "Pos_z_Preview_Road[m]"
  Speed_Limit_Preview_Road[km|h]_/1(Out1) -> Bus Creator/44  "Speed_Limit_Preview_Road[km|h]"
  Curv_Preview_Road[1|m]_/1(Out1) -> Bus Creator/43  "Curv_Preview_Road[1|m]"
  y_Preview_DriverCurv[m]/1 -> y_Preview_DriverCurv[m]_/1(In1)
  x_Preview_DriverCurv[m]/1 -> x_Preview_DriverCurv[m]_/1(In1)
  Pitch_Preview_Road[deg]/1 -> Pitch_Preview_Road[deg]_/1(In1)
  Roll_Preview_Road[deg]/1 -> Roll_Preview_Road[deg]_/1(In1)
  Pos_z_Preview_Road[m]/1 -> Pos_z_Preview_Road[m]_/1(In1)
  Speed_Limit_Preview_Road[km|h]/1 -> Speed_Limit_Preview_Road[km|h]_/1(In1)
  Curv_Preview_Road[1|m]/1 -> Curv_Preview_Road[1|m]_/1(In1)
  s_Total_Vehicle_Road[m]/1 -> s_Total_Vehicle_Road[m]_/1(In1)
  s_Total_Vehicle_Road[m]_/1(Out1) -> Bus Creator/41  "s_Total_Vehicle_Road[m]"
  Reset_VehicleStates[0|1]/1 -> Reset_VehicleStates[0|1]_/1(In1)
  T_Ambient[degC]/1 -> T_Ambient[degC]_/1(In1)
  Reset_VehicleStates[0|1]_/1(Out1) -> Bus Creator/23  "Reset_States[0|1]"
  T_Ambient[degC]_/1(Out1) -> Bus Creator/31  "T_Ambient[degC]"
  p_Ambient[Pa]/1 -> p_Ambient[Pa]_/1(In1)
  p_Ambient[Pa]_/1(Out1) -> Bus Creator/32  "p_Ambient[Pa]"
  ECU_Commands[]_/1(Out1) -> Bus Creator/24  "ECU_Commands[]"
  ECU_Commands[]/1 -> ECU_Commands[]_/1(In1)
  Sw_SteeringMode[1Angle|2Trq]/1 -> Sw_SteeringMode[1Angle|2Trq]_/1(In1)
  q_dt_Vehicle_Init[6x1]_/1(Out1) -> Bus Creator/25  "q_dt_Vehicle_Init[6x1]"
  Trq_Driver_External[Nm]/1 -> Trq_Driver_External[Nm]_/1(In1)
  Pos_Vehicle_Init_CoorSys_E[x;y;z][m]_/1(Out1) -> Bus Creator/36  "Pos_Vehicle_Init_CoorSys_E[x;y;z][m]"
  v_Wind_Coor_Sys_E[x;y;z][m|s]_/1(Out1) -> Bus Creator/38  "v_Wind_Coor_Sys_E[x;y;z][m|s]"
  UnitVec_z_CP[:][x;y;z]/1 -> UnitVec_z_CP[:][x;y;z]_/1(In1)
  Fric_Coeff_CP[:][]/1 -> Fric_Coeff_CP[:][]_/1(In1)
  Sw_SteeringMode[1Angle|2Trq]_/1(Out1) -> Bus Creator/27  "Sw_SteeringMode[1Angle|2Trq]"
  q_dt_Vehicle_Init[6x1]/1 -> q_dt_Vehicle_Init[6x1]_/1(In1)
  Fric_Coeff_CP[:][]_/1(Out1) -> Bus Creator/33  "Fric_Coeff_CP[:][]"
  Pos_z_CP[:][m]_/1(Out1) -> Bus Creator/34  "Pos_z_CP[:][m]"
  Pos_z_CP[:][m]/1 -> Pos_z_CP[:][m]_/1(In1)
  v_Wind_Coor_Sys_E[x;y;z][m|s]/1 -> v_Wind_Coor_Sys_E[x;y;z][m|s]_/1(In1)
  UnitVec_z_CP[:][x;y;z]_/1(Out1) -> Bus Creator/35  "UnitVec_z_CP[:][x;y;z]"
  Angle_Vehicle_Init_CoorSys_E[x;y;z][rad]_/1(Out1) -> Bus Creator/37  "Angle_Vehicle_Init_CoorSys_E[x;y;z][rad]"
  Trq_Driver_External[Nm]_/1(Out1) -> Bus Creator/26  "Trq_Driver_External[Nm]"
  s_Fellows_Ref[m]_/1(Out1) -> Bus Creator/60  "s_Fellows_Ref[m]"
  Angle_Hor_Rel_Fellows[deg]_/1(Out1) -> Bus Creator/58  "Angle_Hor_Rel_Fellows[deg]"
  d_Total_Fellows[m]_/1(Out1) -> Bus Creator/61  "d_Total_Fellows[m]"
  s_Vehicle_Road[m]_/1(Out1) -> Bus Creator/40  "s_Vehicle_Road[m]"
  Length_Fellows[m]_/1(Out1) -> Bus Creator/63  "Length_Fellows[m]"
  Object_ID[]_/1(Out1) -> Bus Creator/59  "Object_ID[]"
  PosVec_MainPnt_Fellows[x;y;z][m]_/1(Out1) -> Bus Creator/62  "PosVec_MainPnt_Fellows[x;y;z][m]"
  Width_Fellows[m]_/1(Out1) -> Bus Creator/64  "Width_Fellows[m]"
  d_Vehicle_Road[m]_/1(Out1) -> Bus Creator/42  "d_Vehicle_Road[m]"
  Width_Fellows[m]/1 -> Width_Fellows[m]_/1(In1)
  Length_Fellows[m]/1 -> Length_Fellows[m]_/1(In1)
  Height_Fellows[m]/1 -> Height_Fellows[m]_/1(In1)
  v_Rel_Fellows[m|s]/1 -> v_Rel_Fellows[m|s]_/1(In1)
  d_Vehicle_Road[m]/1 -> d_Vehicle_Road[m]_/1(In1)
  Dist_Fellows[m]/1 -> Dist_Fellows[m]_/1(In1)
  v_Rel_Fellows[m|s]_/1(Out1) -> Bus Creator/57  "v_Rel_Fellows[m|s]"
  PosVec_MainPnt_Fellows[x;y;z][m]/1 -> PosVec_MainPnt_Fellows[x;y;z][m]_/1(In1)
  s_Vehicle_Road[m]/1 -> s_Vehicle_Road[m]_/1(In1)
  Object_ID[]/1 -> Object_ID[]_/1(In1)
  Angle_Hor_Rel_Fellows[deg]/1 -> Angle_Hor_Rel_Fellows[deg]_/1(In1)
  s_Fellows_Ref[m]/1 -> s_Fellows_Ref[m]_/1(In1)
  d_Total_Fellows[m]/1 -> d_Total_Fellows[m]_/1(In1)
  Height_Fellows[m]_/1(Out1) -> Bus Creator/65  "Height_Fellows[m]"
  Dist_Fellows[m]_/1(Out1) -> Bus Creator/56  "Dist_Fellows[m]"
  Slope_Veh_Road[%]/1 -> Slope_Veh_Road[%]_/1(In1)
  Slope_Veh_Road[%]_/1(Out1) -> Bus Creator/39  "Slope_Veh_Road[%]"
  Pos_Vehicle_Init_CoorSys_E[x;y;z][m]/1 -> Pos_Vehicle_Init_CoorSys_E[x;y;z][m]_/1(In1)
  Angle_Vehicle_Init_CoorSys_E[x;y;z][rad]/1 -> Angle_Vehicle_Init_CoorSys_E[x;y;z][rad]_/1(In1)
  Keep_VehiclePosition[0|1]/1 -> Keep_VehiclePosition[0|1]_/1(In1)
  Sw_Testbench[0Off|1On]/1 -> Sw_Testbench[0Off|1On]_/1(In1)
  Mode_Steer[1Stim|2Driver|3Fix]/1 -> Mode_Steer[1Stim|2Driver|3Fix]_/1(In1)
  Sw_Steering_Mode[1Manual|2ManSched]/1 -> Sw_Steering_Mode[1Manual|2ManSched]_/1(In1)
  Mode_AcceleratorBrake[1Stim|2Driver]/1 -> Mode_AcceleratorBrake[1Stim|2Driver]_/1(In1)
  Mode_GearClutch[1Stim|2Driver|3OpenClutch|4RefGear]/1 -> Mode_GearClutch[1Stim|2Driver|3OpenClutch|4RefGear]_/1(In1)
  Sw_LatDriver[1LatCtrl1|2LatCtrl2]/1 -> Sw_LatDriver[1LatCtrl1|2LatCtrl2]_/1(In1)
  Mode_TrafficDriver[1Off|2On]/1 -> Mode_TrafficDriver[1Off|2On]_/1(In1)
  Mode_LatCtrl[1Pos|2Yaw]/1 -> Mode_LatCtrl[1Pos|2Yaw]_/1(In1)
  Mode_Road[1NoRoad|2Straight|3Circle|4Road]/1 -> Mode_Road[1NoRoad|2Straight|3Circle|4Road]_/1(In1)
  Mode_CurvatureCalculation[1Road|2Driver]_/1(Out1) -> Bus Creator/76  "Mode_CurvatureCalculation[1Road|2Driver]"
  Mode_SelectorLever[1Stim|2Driver]/1 -> Mode_SelectorLever[1Stim|2Driver]_/1(In1)
  Mode_RelativeLane[0CenterLane|1PreferredLane]/1 -> Mode_RelativeLane[0CenterLane|1PreferredLane]_/1(In1)
  Mode_ForceToRoad[1Off|2On]/1 -> Mode_ForceToRoad[1Off|2On]_/1(In1)
  Mode_ForceToRoad[1Off|2On]_/1(Out1) -> Bus Creator/74  "Mode_ForceToRoad[1Off|2On]"
  Mode_AdaptVelocityToRoad[1Off|2On]/1 -> Mode_AdaptVelocityToRoad[1Off|2On]_/1(In1)
  Sw_Testbench[0Off|1On]_/1(Out1) -> Bus Creator/66  "Sw_Testbench[0Off|1On]"
  Mode_StartButtonState[1Stim|2SoftECU]/1 -> Mode_StartButtonState[1Stim|2SoftECU]_/1(In1)
  Sw_LatDriver[1LatCtrl1|2LatCtrl2]_/1(Out1) -> Bus Creator/71  "Sw_LatDriver[1LatCtrl1|2LatCtrl2]"
  Sw_Steering_Mode[1Manual|2ManSched]_/1(Out1) -> Bus Creator/80  "Sw_Steering_Mode[1Manual|2ManSched]"
  Mode_TrafficDriver[1Off|2On]_/1(Out1) -> Bus Creator/77  "Mode_TrafficDriver[1Off|2On]"
  Sw_Tire_Parameter_Set_CP[:][1|2|3|4]_/1(Out1) -> Bus Creator/83  "Sw_Tire_Parameter_Set_CP[:][1|2|3|4]"
  Mode_Road[1NoRoad|2Straight|3Circle|4Road]_/1(Out1) -> Bus Creator/70  "Mode_Road[1NoRoad|2Straight|3Circle|4Road]"
  Mode_StartButtonState[1Stim|2SoftECU]_/1(Out1) -> Bus Creator/79  "Mode_StartButtonState[1Stim|2SoftECU]"
  Mode_AcceleratorBrake[1Stim|2Driver]_/1(Out1) -> Bus Creator/67  "Mode_AcceleratorBrake[1Stim|2Driver]"
  Const_Steering_Mode_Manual[1Angle|2Trq]_/1(Out1) -> Bus Creator/81  "Const_Steering_Mode_Manual[1Angle|2Trq]"
  Mode_SelectorLever[1Stim|2Driver]_/1(Out1) -> Bus Creator/75  "Mode_SelectorLever[1Stim|2Driver]"
  Mode_Steer[1Stim|2Driver|3Fix]_/1(Out1) -> Bus Creator/69  "Mode_Steer[1Stim|2Driver|3Fix]"
  Mode_CurvatureCalculation[1Road|2Driver]/1 -> Mode_CurvatureCalculation[1Road|2Driver]_/1(In1)
  Const_Steering_Mode_Manual[1Angle|2Trq]/1 -> Const_Steering_Mode_Manual[1Angle|2Trq]_/1(In1)
  Keep_VehiclePosition[0|1]_/1(Out1) -> Bus Creator/82  "Keep_VehiclePosition[0|1]"
  Mode_LatCtrl[1Pos|2Yaw]_/1(Out1) -> Bus Creator/72  "Mode_LatCtrl[1Pos|2Yaw]"
  Mode_GearClutch[1Stim|2Driver|3OpenClutch|4RefGear]_/1(Out1) -> Bus Creator/68  "Mode_GearClutch[1Stim|2Driver|3OpenClutch|4RefGear]"
  Mode_RelativeLane[0CenterLane|1PreferredLane]_/1(Out1) -> Bus Creator/78  "Mode_RelativeLane[0CenterLane|1PreferredLane]"
  Sw_Tire_Parameter_Set_CP[:][1|2|3|4]/1 -> Sw_Tire_Parameter_Set_CP[:][1|2|3|4]_/1(In1)
  Mode_AdaptVelocityToRoad[1Off|2On]_/1(Out1) -> Bus Creator/73  "Mode_AdaptVelocityToRoad[1Off|2On]"
  Activate_DCLink[0Off|1On]_/1(Out1) -> Bus Creator/87  "Activate_DCLink[0Off|1On]"
  I_Load_LV[A]_/1(Out1) -> Bus Creator/89  "I_Load_LV[A]"
  I_Load_LV[A]/1 -> I_Load_LV[A]_/1(In1)
  Activate_DCLink[0Off|1On]/1 -> Activate_DCLink[0Off|1On]_/1(In1)
  I_Load_HV[A]/1 -> I_Load_HV[A]_/1(In1)
  I_Load_HV[A]_/1(Out1) -> Bus Creator/88  "I_Load_HV[A]"

== system ASM_Traffic_A11/Environment/Maneuver/PlantModel ==
  UserInterface : Inport
  In : Inport  Port=2
  ASMSignalCollector : Subsystem
  AvoidAlgLoop{,1..3,5..9} (9 alike) : UnitDelay  SampleTime=-1
  Bus Selector : BusSelector  OutputSignals=Plant.Road_Info.RoadState[],Plant.Road_ASMVeh.s_Veh_Road[m],Plant.Road_ASMVeh.s_Total_Veh_Road[m],Plant.Road_ASMVeh.s_Veh_Road_Trj[m],Plant.Road_Info.Dist_Response_Maneuver.Distance_xy[m]
  Bus Selector1 : BusSelector  OutputSignals=ExternalModel.s_Vehicle[m],ExternalModel.v_x_Vehicle_CoG[km|h],ExternalModel.a_y_Vehicle_CoG[m|s2],ExternalModel.Const_r_unloaded_Tire_Mean[m]
  Bus Selector10 : BusSelector  OutputSignals=Interface_In
  Bus Selector11 : BusSelector  OutputSignals=Sw_ManeuverSelect[1_6],Sw_ManeuverSettings
  Bus Selector12 : BusSelector  OutputSignals=Interface_In
  Bus Selector13 : BusSelector  OutputSignals=ManualControl.ManualDriving.Pos_AccPedal[%],ManualControl.ManualDriving.Pos_BrakePedal[%],ManualControl.ManualDriving.Pos_ClutchPedal[%],ManualControl.ManualDriving.Gear[],ManualControl.ManualDriving.Angle_SteeringWheel[deg],ManualControl.ManualDriving.v_Vehicle_Ref[m|s],ManualControl.ManualDriving.d_Ref[m],ManualControl.ManualDriving.LaneIdx_Ref[],ManualControl.ManualDriving.Trq_Steering[Nm],ManualControl.ManualDriving.SelectorLever[]  OutputAsBus=on
  Bus Selector2 : BusSelector  OutputSignals=GroundTruth
  Bus Selector3 : BusSelector  OutputSignals=Road
  Bus Selector4 : BusSelector  OutputSignals=Traffic
  Bus Selector5 : BusSelector  OutputSignals=ManeuverState[]
  Bus Selector6 : BusSelector  OutputSignals=ExternalModel.t_Preview_vRef_Driver[s]
  Bus Selector7 : BusSelector  OutputSignals=Plant.Traffic_Signals_toEnvironment.Dist_Refline_Response[m]
  Bus Selector8 : BusSelector  OutputSignals=Sw_ManeuverControl.ManeuverStart[0|1],Sw_ManeuverControl.ManeuverStop[0|1],Sw_ManeuverControl.Sw_ManualDriving[1ManSched|2Manual]  OutputAsBus=on
  Bus Selector9 : BusSelector  OutputSignals=Plant.Control.Interface_Init_Ready[0Off|1On]
  Bus to Vector : BusToVector
  Customize_UserSignals : Subsystem
  Demux3 : Demux  Outputs=3
      settings: DisplayOption=none
  ExternalSegmentEnd : Subsystem
  ExternalUserData : Subsystem
  Goto Tag Visibility : GotoTagVisibility  GotoTag=ASMBUS_Environment_ManeuverScheduler
  Goto Tag Visibility1 : GotoTagVisibility  GotoTag=ASMBUS_Environment_Mnvr_UserSignalsCustomized
  InitialVehicleStates : Subsystem
  LastValues : Subsystem
  MANEUVER_SCHEDULER : ASM_Environment_lib/Environment/Maneuver/MANEUVER_SCHEDULER  Tag=ASM_SUBCOMPONENT  Maneuver_ModelDesk=MDL.Environment.Maneuver.Maneuver_ModelDesk  Maneuver_2=MDL.Environment.Maneuver.Maneuver_2  Maneuver_3=MDL.Environment.Maneuver.Maneuver_3  Maneuver_4=MDL.Environment.Maneuver.Maneuver_4  Maneuver_5=MDL.Environment.Maneuver.Maneuver_5  Maneuver_6=MDL.Environment.Maneuver.Maneuver_6  StepSize=SIM.StepSize  ASMProperties=struct('Name','MANEUVER_SCHEDULER','Version','27.0','Library','ASM_Environment_lib')  ASMInstanceName=maneuver_scheduler  ASMInstanceID=1
  MANEUVER_STATE : ASM_Utils_lib/ModelDeskInterface/ManeuverControl/MANEUVER_STATE  Tag=ASM_SUBCOMPONENT  ASMProperties=struct('Name','MANEUVER_STATE','Version','1.0','Library','ASM_Utils_lib')  ASMInstanceName=maneuver_state  ASMInstanceID=1
  MODEL_DESK_WRITE_ACCESS : ASM_Utils_lib/ModelDeskInterface/MODEL_DESK_WRITE_ACCESS  Tag=ASM_SUBCOMPONENT  ASMProperties=struct('Name','MODEL_DESK_WRITE_ACCESS','Version','1.0','Library','ASM_Utils_lib')  ModelDesk_WriteAccess=MDL.Environment.ModelDesk_WriteAccess  ASMInstanceName=model_desk_write_access  ASMInstanceID=1
  ManeuverReset : Subsystem
  ROADSTATE_RUN_TRIGGER : ASM_Environment_lib/Environment/Maneuver/ROADSTATE_RUN_TRIGGER  ASMProperties=struct('Name','ROADSTATE_RUN_TRIGGER','Version','1.0','Library','ASM_Environment_lib')  ASMInstanceName=roadstate_run_trigger  ASMInstanceID=1
  ReplaceBrake : Subsystem
  ReplaceSelectorLever_Mode : Subsystem
  SimulationControl : Subsystem
  Terminator : Terminator
  UnitConversion : ASM_Utils_lib/UnitConversion/UnitConversion  Selection=km/h_to_m/s
  ASMSignalBus : Outport  VectorParamsAs1DForOutWhenUnconnected=off
  tag scope: ASMBUS_Environment_ManeuverScheduler=scoped, ASMBUS_Environment_Mnvr_UserSignalsCustomized=scoped
  wires:
  ManeuverReset/1(Reset[0|1]) -> MANEUVER_SCHEDULER/6
  Customize_UserSignals/2(UserSignals_Customized) -> ExternalSegmentEnd/2(UserSignals_Customized)
  AvoidAlgLoop1/1 -> MANEUVER_SCHEDULER/17
  ExternalSegmentEnd/1(External_SegmentEnd[0|1]) -> MANEUVER_SCHEDULER/22
  Bus Selector1/3 -> AvoidAlgLoop/1  "<a_y_Vehicle_CoG[m|s2]>"
  Bus Selector/3 -> AvoidAlgLoop5/1  "<s_Total_Veh_Road[m]>"
  MANEUVER_SCHEDULER/5 -> LastValues/2(Maneuver_RefSignals), ReplaceBrake/2(RefSignals_In)
  AvoidAlgLoop3/1 -> MANEUVER_SCHEDULER/11
  AvoidAlgLoop6/1 -> MANEUVER_SCHEDULER/19
  AvoidAlgLoop7/1 -> MANEUVER_SCHEDULER/14
  SimulationControl/1(Keep_VehiclePosition[0|1]) -> MANEUVER_SCHEDULER/7
  AvoidAlgLoop5/1 -> MANEUVER_SCHEDULER/12
  MANEUVER_SCHEDULER/6 -> Terminator/1
  Bus Selector1/2 -> UnitConversion/1  "<v_x_Vehicle_CoG[km|h]>"
  Bus Selector6/1 -> AvoidAlgLoop8/1  "<t_Preview_vRef_Driver[s]>"
  LastValues/1(LastValues) -> MANEUVER_SCHEDULER/9
  AvoidAlgLoop8/1 -> MANEUVER_SCHEDULER/23
  MANEUVER_SCHEDULER/8 -> Customize_UserSignals/1(UserSignals_In)
  Bus Selector7/1 -> MANEUVER_SCHEDULER/15  "<Dist_Refline_Response[m]>"
  Bus Selector/5 -> AvoidAlgLoop7/1  "<Distance_xy[m]>"
  Bus Selector1/1 -> AvoidAlgLoop2/1  "<s_Vehicle[m]>"
  Bus Selector13/1 -> MANEUVER_SCHEDULER/20
  Customize_UserSignals/1(ASMSignalBus) -> [ASMBUS_Environment_Mnvr_UserSignalsCustomized]
  MANEUVER_SCHEDULER/2 -> InitialVehicleStates/2(MdlControl)
  AvoidAlgLoop/1 -> MANEUVER_SCHEDULER/18
  MANEUVER_SCHEDULER/3 -> InitialVehicleStates/3(InitialVehStates)
  AvoidAlgLoop2/1 -> MANEUVER_SCHEDULER/16
  ROADSTATE_RUN_TRIGGER/1 -> MANEUVER_SCHEDULER/10
  MODEL_DESK_WRITE_ACCESS/1 -> MANEUVER_SCHEDULER/8
  Bus Selector/4 -> AvoidAlgLoop9/1  "<s_Veh_Road_Trj[m]>"
  UnitConversion/1 -> AvoidAlgLoop1/1
  Bus Selector5/1 -> MANEUVER_STATE/1  "<ManeuverState[]>"
  MANEUVER_SCHEDULER/7 -> Bus Selector5/1, ReplaceBrake/3(Info[]), InitialVehicleStates/4(Info[])
  ExternalUserData/1(External_ReferenceSignals) -> MANEUVER_SCHEDULER/21
  In/1 -> ManeuverReset/2(In), SimulationControl/2(In), Bus Selector3/1, Bus Selector4/1, Bus Selector10/1, ExternalSegmentEnd/1(In), Bus Selector12/1, Bus Selector2/1, LastValues/1(In), ReplaceBrake/1(In)
  InitialVehicleStates/1(VehicleInitStates) -> ASMSignalCollector/2(VehicleInitStates)
  Bus Selector1/4 -> AvoidAlgLoop6/1  "<Const_r_unloaded_Tire_Mean[m]>"
  MANEUVER_SCHEDULER/1 -> [ASMBUS_Environment_ManeuverScheduler]
  AvoidAlgLoop9/1 -> MANEUVER_SCHEDULER/13
  ReplaceBrake/1(RefSignals) -> ASMSignalCollector/4(RefSignals)
  Bus Selector9/1 -> ROADSTATE_RUN_TRIGGER/1  "<Interface_Init_Ready[0Off|1On]>"
  Bus Selector/2 -> AvoidAlgLoop3/1  "<s_Veh_Road[m]>"
  ReplaceSelectorLever_Mode/1(ModeSignals) -> ASMSignalCollector/3(ModeSignals)
  MANEUVER_SCHEDULER/4 -> ReplaceSelectorLever_Mode/2(ModeSignals_In)
  ASMSignalCollector/1(Maneuver_Signals) -> ASMSignalBus/1  "Plant"
  InitialVehicleStates/2(Flag_Init_Drivetrain[0InProgress|1Finished]) -> MANEUVER_SCHEDULER/24
  UserInterface/1 -> ManeuverReset/1(UserInterface), Bus Selector13/1, SimulationControl/1(UserInterface), Bus Selector8/1, Bus Selector11/1, ASMSignalCollector/1(UserInterface), InitialVehicleStates/1(UserInterface), ReplaceSelectorLever_Mode/1(UserInterface)
  Bus Selector11/1 -> MANEUVER_SCHEDULER/1  "<Sw_ManeuverSelect[1_6]>"
  Bus Selector11/2 -> MANEUVER_SCHEDULER/2  "<Sw_ManeuverSettings>"
  Bus Selector8/1 -> Bus to Vector/1
  Bus to Vector/1 -> Demux3/1
  Demux3/1 -> MANEUVER_SCHEDULER/3
  Demux3/2 -> MANEUVER_SCHEDULER/4
  Demux3/3 -> MANEUVER_SCHEDULER/5
  Bus Selector/1 -> ROADSTATE_RUN_TRIGGER/2  "<RoadState[]>"
  Bus Selector2/1 -> Bus Selector9/1  "<GroundTruth>"
  Bus Selector3/1 -> Bus Selector/1  "<Road>"
  Bus Selector4/1 -> Bus Selector7/1  "<Traffic>"
  Bus Selector10/1 -> Bus Selector1/1  "<Interface_In>"
  Bus Selector12/1 -> Bus Selector6/1  "<Interface_In>"

== system ASM_Traffic_A11/Environment/Maneuver/UserInterface ==
  note: Maneuver
  Interface_In : Inport
  In : Inport  Port=2
  ASMSignalBus_Plant : Subsystem
  DISP_Plant : Subsystem
  PAR_Plant : Subsystem
  Out : Outport  VectorParamsAs1DForOutWhenUnconnected=off
  wires:
  In/1 -> DISP_Plant/1(In), ASMSignalBus_Plant/1(In)
  Interface_In/1 -> PAR_Plant/1(Interface_In)
  PAR_Plant/1(Out) -> Out/1
